simulink model "b0_min"  (R2023b)
settings: Solver=FixedStepDiscrete  StartTime=0.0  StopTime=12  FixedStep=0.001  RelTol=1e-3
settings Model: Creator=28447  LastModifiedBy=28447
settings SFSimCC: SimCustomHeaderCode=extern void b0_ident_u(const float in[5], float out[2]);  SimUserIncludeDirs=D:\Desktop\RCESO\simulink
settings SFSimCC: SimUserSources=|
  | D:\Desktop\RCESO\simulink\b0_ident.c
  | D:\Desktop\RCESO\simulink\b0_ident_wrap.c
settings RTWCC: CustomSource=|
  | D:\Desktop\RCESO\simulink\b0_ident.c
  | D:\Desktop\RCESO\simulink\b0_ident_wrap.c

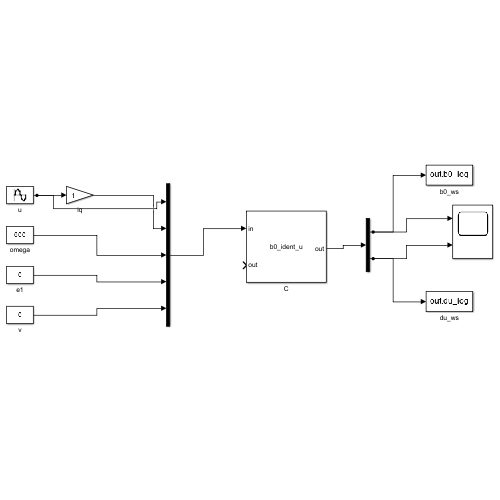
[thumbnail: Simulink's stored preview of the top-level diagram]
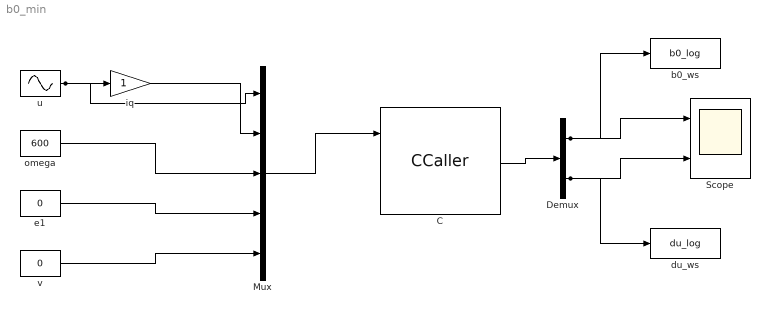
== system b0_min ==
  C : CCaller  FunctionName=b0_ident_u  PortSpecificationStruct="%)30     .    P ,   8    (     @         %    \"     (    !     0         %  0 \"0    $    _    07)G3F%M90  4&]R=$YA;64 4V-O<&4     26YD97@     5'EP90      4VEZ90      27-';&]B86P   X    P    !@    @    $          4    (     0    (    !         !   @!I;@  #@   #     &    \"     0         !0    @    !     @    $         $  \" &EN   .    .     8    (    !          %    \"     $    %     0         0    !0   $EN<'5T    #@   #@    &    \"     8         !0    @    !     0    $         \"0    @               X    X    !@    @    $          4    (     0    8    !         !     &    <VEN9VQE   .    ,     8    (    !          %    \"     $    !     0         0  $ -0    X    P    !@    @    ) @        4    (     0    $    !          (  0      #@   #     &    \"     0         !0    @    !     P    $         $  # &]U=  .    ,     8    (    !          %    \"     $    #     0         0  , ;W5T  X   !     !@    @    $          4    (     0    L    !         !     +    26YP=71/=71P=70       X    X    !@    @    &          4    (     0    $    !          D    (            \\#\\.    .     8    (    !          %    \"     $    &     0         0    !@   '-I;F=L90  #@   #     &    \"     0         !0    @    !     0    $         $  ! #(    .    ,     8    (    \"0(        %    \"     $    !     0         \"  $"
  Demux : Demux  Outputs=2
  Mux : Mux  Inputs=5
  Scope : Scope  NumInputPorts=2
  b0_ws : ToWorkspace  VariableName=b0_log  SaveFormat=Timeseries  SampleTime=0.001
  du_ws : ToWorkspace  VariableName=du_log  SaveFormat=Timeseries  SampleTime=0.001
  e1 : Constant  Value=0  SampleTime=0.001
  iq : Gain
  omega : Constant  Value=600  SampleTime=0.001
  u : Sin  Amplitude=0.118  Frequency=2*pi*65  SampleTime=0.001
  v : Constant  Value=0  SampleTime=0.001
  wires:
  u/1 -> iq/1, Mux/1
  iq/1 -> Mux/2
  omega/1 -> Mux/3
  e1/1 -> Mux/4
  v/1 -> Mux/5
  Mux/1 -> C/1
  C/1 -> Demux/1
  Demux/1 -> Scope/1, b0_ws/1
  Demux/2 -> Scope/2, du_ws/1
